simulink model "F90_XMED_03"  (R2025a)
settings: Solver=VariableStepAuto  StartTime=0.0  StopTime=24  RelTol=1e-3
model workspace (MATLAB code in the model file):
  | v_M_exhale = 490; % cmH2O (PEEP)
  | v_M_inhale = 1471; % (PIP)
  | R_M = 0; %
  | 
  | R_V1 = 5670; % cmH2O/L/s
  | R_V2 = 5670;
  | R_I1 = 5670; % tube length = 1.8 ms
  | R_I2 = 5670;
  | R_EV1 = 0;
  | R_EV2 = 0;
  | 
  | R_L1 = 196133;
  | R_L2 = 196133;
  | C_L1 = 5.50647e-7; % L/cmH2O
  | C_L2 = 5.50647e-7;
  | R_ETT1 = 784000;
  | R_ETT2 = 784000;
  | 
  | % === artificial patients (bags)s ====
  | R_aL1 = 196133;
  | R_aL2 = 196133;
  | C_aL1 = 5.50647e-7;
  | C_aL2 = 5.50647e-7;
  | % =======
  | 
  | R_E1 = 5670;
  | R_E2 = 5670;
  | R_O = 0;
  | 
  | RR = 15;
  | I = 1;
  | E = 2;
  | IE_ratio = I/ E;
undefined symbols (not defined in the file): max_inspiratory_pressure_cmH2O, patient1_compliance_L_per_cmH2O, patient1_resistance_cmH2O_per_Lps, patient2_compliance_L_per_cmH2O, patient2_resistance_cmH2O_per_Lps, peep_cmH2O, respiratory_rate_bpm, target_step_time_s, target_tv1_final_mL, target_tv1_initial_mL, target_tv2_final_mL, target_tv2_initial_mL
libraries: fl_lib x39, nesl_utility x16
settings Model: Creator=jsolislemus  LastModifiedBy=SimuVerity Contributors
settings SolverCC: AlgebraicLoopSolver=TrustRegion
settings DataIOCC: SignalLogging=off
settings DebuggingCC: UnconnectedInputMsg=warning  UnconnectedOutputMsg=warning  UnconnectedLineMsg=warning
settings ModelReferenceCC: EnableRefExpFcnMdlSchedulingChecks=on
settings RTWCC: GPUComputeCapability=3.5

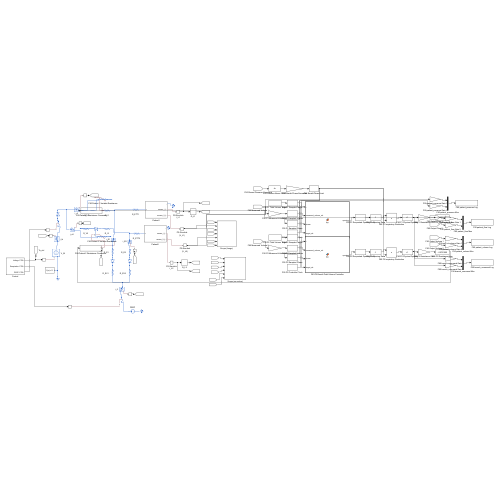
[thumbnail: Simulink's stored preview of the top-level diagram]
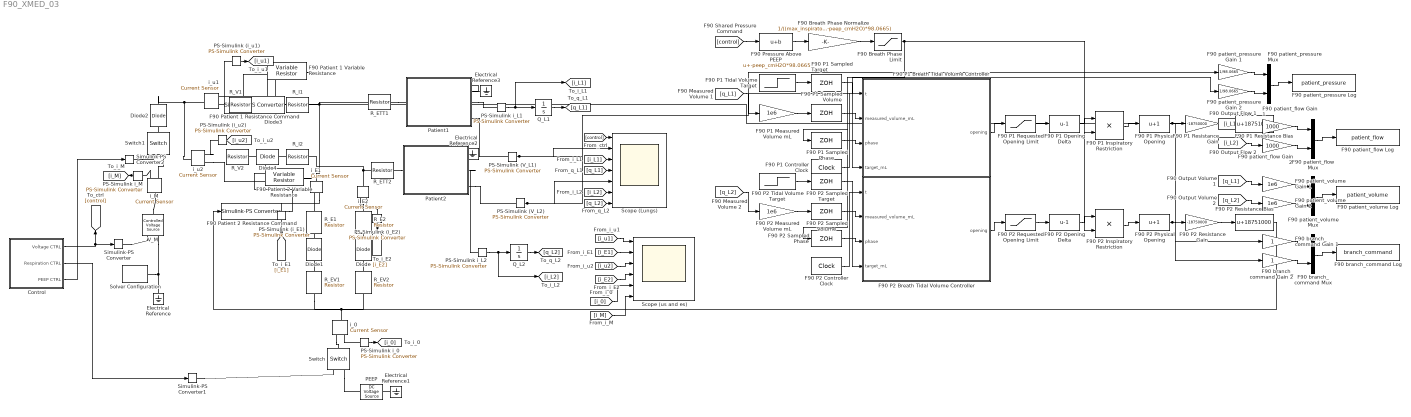
== system F90_XMED_03 ==
  Control : Subsystem
  Diode{,1..4} (5 alike) : fl_lib/Electrical/Electrical Elements/Diode  Vf=0.6 V  Ron=0.3 Ohm  Goff=1e-8 1/Ohm  i_specify=off  i_priority=None  i=0 A  i_nominal_specify=off  i_nominal_value=1  i_nominal_unit=A  v_specify=off  v_priority=None  v=0 V  v_nominal_specify=off  v_nominal_value=1  v_nominal_unit=V
  Electrical Reference{,1..3} (4 alike) : fl_lib/Electrical/Electrical Elements/Electrical Reference
  F90 Breath Phase Limit : Saturate  UpperLimit=1  LowerLimit=0
  F90 Breath Phase Normalize : Gain  Gain=1/((max_inspiratory_pressure_cmH2O-peep_cmH2O)*98.0665)
  F90 P1 Breath Tidal Volume Controller : MATLAB Function  TreatAsAtomicUnit=on
  F90 P1 Controller Clock : DigitalClock  SampleTime=0.005
  F90 P1 Inspiratory Restriction : Product  Inputs=**
  F90 P1 Measured Volume mL : Gain  Gain=1e6
  F90 P1 Opening Delta : Bias  Bias=-1  SaturateOnIntegerOverflow=off
  F90 P1 Physical Opening : Bias  Bias=1  SaturateOnIntegerOverflow=off
  F90 P1 Requested Opening Limit : Saturate  UpperLimit=1  LowerLimit=0.02
  F90 P1 Resistance Bias : Bias  Bias=18751000  SaturateOnIntegerOverflow=off
  F90 P1 Resistance Gain : Gain  Gain=-18750000
  F90 P1 Sampled Phase : ZeroOrderHold  SampleTime=0.005
  F90 P1 Sampled Target : ZeroOrderHold  SampleTime=0.005
  F90 P1 Sampled Volume : ZeroOrderHold  SampleTime=0.005
  F90 P1 Tidal Volume Target : Step  Time=target_step_time_s  Before=target_tv1_initial_mL  After=target_tv1_final_mL  SampleTime=0
  F90 P2 Breath Tidal Volume Controller : MATLAB Function  TreatAsAtomicUnit=on
  F90 P2 Controller Clock : DigitalClock  SampleTime=0.005
  F90 P2 Inspiratory Restriction : Product  Inputs=**
  F90 P2 Measured Volume mL : Gain  Gain=1e6
  F90 P2 Opening Delta : Bias  Bias=-1  SaturateOnIntegerOverflow=off
  F90 P2 Physical Opening : Bias  Bias=1  SaturateOnIntegerOverflow=off
  F90 P2 Requested Opening Limit : Saturate  UpperLimit=1  LowerLimit=0.02
  F90 P2 Resistance Bias : Bias  Bias=18751000  SaturateOnIntegerOverflow=off
  F90 P2 Resistance Gain : Gain  Gain=-18750000
  F90 P2 Sampled Phase : ZeroOrderHold  SampleTime=0.005
  F90 P2 Sampled Target : ZeroOrderHold  SampleTime=0.005
  F90 P2 Sampled Volume : ZeroOrderHold  SampleTime=0.005
  F90 P2 Tidal Volume Target : Step  Time=target_step_time_s  Before=target_tv2_initial_mL  After=target_tv2_final_mL  SampleTime=0
  F90 Patient 1 Resistance Command : nesl_utility/Simulink-PS Converter  PhysicalDomain=network_engine_domain  SubClassName=ps_input  LeftPortType=input  RightPortType=output  PseudoPeriodic=off  Frequencies=[]  NoiseDistribution=none  NoiseParameters=[]  Unit=Ohm  AffineConversion=off  FilteringAndDerivatives=filter  SimscapeFilterOrder=1  InputFilterTimeConstant=0.002  UdotUserProvided=0
  F90 Patient 1 Variable Resistance : fl_lib/Electrical/Electrical Elements/Variable Resistor  Rmin=1 Ohm  thermalEnable=false  thermal_mass=1 J/K  i_specify=off  i_priority=None  i=0 A  i_nominal_specify=off  i_nominal_value=1  i_nominal_unit=A  v_specify=off  v_priority=None  v=0 V  v_nominal_specify=off  v_nominal_value=1  v_nominal_unit=V  T_specify=off  T_priority=None  T=300 K  T_nominal_specify=off  T_nominal_value=1  T_nominal_unit=K
  F90 Patient 2 Resistance Command : nesl_utility/Simulink-PS Converter  PhysicalDomain=network_engine_domain  SubClassName=ps_input  LeftPortType=input  RightPortType=output  PseudoPeriodic=off  Frequencies=[]  NoiseDistribution=none  NoiseParameters=[]  Unit=Ohm  AffineConversion=off  FilteringAndDerivatives=filter  SimscapeFilterOrder=1  InputFilterTimeConstant=0.002  UdotUserProvided=0
  F90 Patient 2 Variable Resistance : fl_lib/Electrical/Electrical Elements/Variable Resistor  Rmin=1 Ohm  thermalEnable=false  thermal_mass=1 J/K  i_specify=off  i_priority=None  i=0 A  i_nominal_specify=off  i_nominal_value=1  i_nominal_unit=A  v_specify=off  v_priority=None  v=0 V  v_nominal_specify=off  v_nominal_value=1  v_nominal_unit=V  T_specify=off  T_priority=None  T=300 K  T_nominal_specify=off  T_nominal_value=1  T_nominal_unit=K
  F90 Pressure Above PEEP : Bias  Bias=-peep_cmH2O*98.0665  SaturateOnIntegerOverflow=off
  F90 branch_command Gain 1 : Gain
  F90 branch_command Gain 2 : Gain
  F90 branch_command Log : ToWorkspace  VariableName=branch_command  SaveFormat=Timeseries  SampleTime=-1
  F90 branch_command Mux : Mux  Inputs=2
  F90 patient_flow Gain 1 : Gain  Gain=1000
  F90 patient_flow Gain 2 : Gain  Gain=1000
  F90 patient_flow Log : ToWorkspace  VariableName=patient_flow  SaveFormat=Timeseries  SampleTime=-1
  F90 patient_flow Mux : Mux  Inputs=2
  F90 patient_pressure Gain 1 : Gain  Gain=1/98.0665
  F90 patient_pressure Gain 2 : Gain  Gain=1/98.0665
  F90 patient_pressure Log : ToWorkspace  VariableName=patient_pressure  SaveFormat=Timeseries  SampleTime=-1
  F90 patient_pressure Mux : Mux  Inputs=2
  F90 patient_volume Gain 1 : Gain  Gain=1e6
  F90 patient_volume Gain 2 : Gain  Gain=1e6
  F90 patient_volume Log : ToWorkspace  VariableName=patient_volume  SaveFormat=Timeseries  SampleTime=-1
  F90 patient_volume Mux : Mux  Inputs=2
  PEEP : fl_lib/Electrical/Electrical Sources/DC Voltage Source  v0=v_M_exhale V
  PS-Simulink (V_L1) : nesl_utility/PS-Simulink Converter  PhysicalDomain=network_engine_domain  SubClassName=ps_output  LeftPortType=input  RightPortType=output  PseudoPeriodic=off  Frequencies=[]  VectorFormat=1-D array  Unit=inherit  AffineConversion=off
  PS-Simulink (V_L2) : nesl_utility/PS-Simulink Converter  PhysicalDomain=network_engine_domain  SubClassName=ps_output  LeftPortType=input  RightPortType=output  PseudoPeriodic=off  Frequencies=[]  VectorFormat=1-D array  Unit=inherit  AffineConversion=off
  PS-Simulink (i_E1) : nesl_utility/PS-Simulink Converter  PhysicalDomain=network_engine_domain  SubClassName=ps_output  LeftPortType=input  RightPortType=output  PseudoPeriodic=off  Frequencies=[]  VectorFormat=1-D array  Unit=inherit  AffineConversion=off
  PS-Simulink (i_E2) : nesl_utility/PS-Simulink Converter  PhysicalDomain=network_engine_domain  SubClassName=ps_output  LeftPortType=input  RightPortType=output  PseudoPeriodic=off  Frequencies=[]  VectorFormat=1-D array  Unit=inherit  AffineConversion=off
  PS-Simulink (i_u1) : nesl_utility/PS-Simulink Converter  PhysicalDomain=network_engine_domain  SubClassName=ps_output  LeftPortType=input  RightPortType=output  PseudoPeriodic=off  Frequencies=[]  VectorFormat=1-D array  Unit=inherit  AffineConversion=off
  PS-Simulink (i_u2) : nesl_utility/PS-Simulink Converter  PhysicalDomain=network_engine_domain  SubClassName=ps_output  LeftPortType=input  RightPortType=output  PseudoPeriodic=off  Frequencies=[]  VectorFormat=1-D array  Unit=inherit  AffineConversion=off
  PS-Simulink i_0 : nesl_utility/PS-Simulink Converter  PhysicalDomain=network_engine_domain  SubClassName=ps_output  LeftPortType=input  RightPortType=output  PseudoPeriodic=off  Frequencies=[]  VectorFormat=1-D array  Unit=inherit  AffineConversion=off
  PS-Simulink i_L1 : nesl_utility/PS-Simulink Converter  PhysicalDomain=network_engine_domain  SubClassName=ps_output  LeftPortType=input  RightPortType=output  PseudoPeriodic=off  Frequencies=[]  VectorFormat=1-D array  Unit=inherit  AffineConversion=off
  PS-Simulink i_L2 : nesl_utility/PS-Simulink Converter  PhysicalDomain=network_engine_domain  SubClassName=ps_output  LeftPortType=input  RightPortType=output  PseudoPeriodic=off  Frequencies=[]  VectorFormat=1-D array  Unit=inherit  AffineConversion=off
  PS-Simulink i_M : nesl_utility/PS-Simulink Converter  PhysicalDomain=network_engine_domain  SubClassName=ps_output  LeftPortType=input  RightPortType=output  PseudoPeriodic=off  Frequencies=[]  VectorFormat=1-D array  Unit=inherit  AffineConversion=off
  Patient1 : Subsystem
  Patient2 : Subsystem
  Q_L1 : Integrator
  Q_L2 : Integrator
  R_E1 : fl_lib/Electrical/Electrical Elements/Resistor  R=R_E1 Ohm  i_specify=off  i_priority=None  i=0 A  i_nominal_specify=off  i_nominal_value=1  i_nominal_unit=A  v_specify=off  v_priority=None  v=0 V  v_nominal_specify=off  v_nominal_value=1  v_nominal_unit=V
  R_E2 : fl_lib/Electrical/Electrical Elements/Resistor  R=R_E2 Ohm  i_specify=off  i_priority=None  i=0 A  i_nominal_specify=off  i_nominal_value=1  i_nominal_unit=A  v_specify=off  v_priority=None  v=0 V  v_nominal_specify=off  v_nominal_value=1  v_nominal_unit=V
  R_ETT1 : fl_lib/Electrical/Electrical Elements/Resistor  R=R_ETT1 Ohm  i_specify=off  i_priority=None  i=0 A  i_nominal_specify=off  i_nominal_value=1  i_nominal_unit=A  v_specify=off  v_priority=None  v=0 V  v_nominal_specify=off  v_nominal_value=1  v_nominal_unit=V
  R_ETT2 : fl_lib/Electrical/Electrical Elements/Resistor  R=R_ETT2 Ohm  i_specify=off  i_priority=None  i=0 A  i_nominal_specify=off  i_nominal_value=1  i_nominal_unit=A  v_specify=off  v_priority=None  v=0 V  v_nominal_specify=off  v_nominal_value=1  v_nominal_unit=V
  R_EV1 : fl_lib/Electrical/Electrical Elements/Resistor  R=R_EV1 Ohm  i_specify=off  i_priority=None  i=0 A  i_nominal_specify=off  i_nominal_value=1  i_nominal_unit=A  v_specify=off  v_priority=None  v=0 V  v_nominal_specify=off  v_nominal_value=1  v_nominal_unit=V
  R_EV2 : fl_lib/Electrical/Electrical Elements/Resistor  R=R_EV2 Ohm  i_specify=off  i_priority=None  i=0 A  i_nominal_specify=off  i_nominal_value=1  i_nominal_unit=A  v_specify=off  v_priority=None  v=0 V  v_nominal_specify=off  v_nominal_value=1  v_nominal_unit=V
  R_I1 : fl_lib/Electrical/Electrical Elements/Resistor  R=R_I1 Ohm  i_specify=off  i_priority=None  i=0 A  i_nominal_specify=off  i_nominal_value=1  i_nominal_unit=A  v_specify=off  v_priority=None  v=0 V  v_nominal_specify=off  v_nominal_value=1  v_nominal_unit=V
  R_I2 : fl_lib/Electrical/Electrical Elements/Resistor  R=R_I2 Ohm  i_specify=off  i_priority=None  i=0 A  i_nominal_specify=off  i_nominal_value=1  i_nominal_unit=A  v_specify=off  v_priority=None  v=0 V  v_nominal_specify=off  v_nominal_value=1  v_nominal_unit=V
  R_V1 : fl_lib/Electrical/Electrical Elements/Resistor  R=R_V1 Ohm  i_specify=off  i_priority=None  i=0 A  i_nominal_specify=off  i_nominal_value=1  i_nominal_unit=A  v_specify=off  v_priority=None  v=0 V  v_nominal_specify=off  v_nominal_value=1  v_nominal_unit=V
  R_V2 : fl_lib/Electrical/Electrical Elements/Resistor  R=R_V2 Ohm  i_specify=off  i_priority=None  i=0 A  i_nominal_specify=off  i_nominal_value=1  i_nominal_unit=A  v_specify=off  v_priority=None  v=0 V  v_nominal_specify=off  v_nominal_value=1  v_nominal_unit=V
  Scope (Lungs) : Scope  NumInputPorts=7
      settings: ActiveDisplayYMinimum=306.25  ActiveDisplayYMaximum=2143.75
  Scope (us and es) : Scope  NumInputPorts=6
      settings: ActiveDisplayYMinimum=-0.00219  ActiveDisplayYMaximum=0.02286  DataLoggingVariableName=ScopeAdvanced
  Simulink-PS Converter : nesl_utility/Simulink-PS Converter  PhysicalDomain=network_engine_domain  SubClassName=ps_input  LeftPortType=input  RightPortType=output  PseudoPeriodic=off  Frequencies=[]  NoiseDistribution=none  NoiseParameters=[]  Unit=1  AffineConversion=off  FilteringAndDerivatives=provide  SimscapeFilterOrder=1  InputFilterTimeConstant=0.001  UdotUserProvided=0
  Simulink-PS Converter1 : nesl_utility/Simulink-PS Converter  PhysicalDomain=network_engine_domain  SubClassName=ps_input  LeftPortType=input  RightPortType=output  PseudoPeriodic=off  Frequencies=[]  NoiseDistribution=none  NoiseParameters=[]  Unit=1  AffineConversion=off  FilteringAndDerivatives=provide  SimscapeFilterOrder=1  InputFilterTimeConstant=0.001  UdotUserProvided=0
  Simulink-PS Converter2 : nesl_utility/Simulink-PS Converter  PhysicalDomain=network_engine_domain  SubClassName=ps_input  LeftPortType=input  RightPortType=output  PseudoPeriodic=off  Frequencies=[]  NoiseDistribution=none  NoiseParameters=[]  Unit=1  AffineConversion=off  FilteringAndDerivatives=provide  SimscapeFilterOrder=1  InputFilterTimeConstant=0.001  UdotUserProvided=0
  Solver Configuration : nesl_utility/Solver Configuration  PhysicalDomain=network_engine_domain  SubClassName=solver  LeftPortType=input  RightPortType=generic  Tones=[]  Harmonics=[]  SimulateNoise=off  Profile=off  UseLocalSampling=off  EnableSwitchedLinearOptims=on  FrequencyDomain=off  UseCCode=off  RelTol=0.001  AbsTol=1e-06  MinStep=1e-09  ToWorkspace=off  RevertToSquareIcSolve=off  NumHomotopyIterations=100  PhasorMode=off  PhasorModeNumHarmonics=1  ConsistencySolver=NEWTON_FTOL  IndexReductionMethod=DerivativeReplacement  DoDC=off  ResidualTolerance=1e-09  ConsistencyTolSource=GLOBAL  ConsistencyAbsTol=0.001  ConsistencyRelTol=0.001  ConsistencyTolFactor=0.001  UseLocalSolver=off  LocalSolverChoice=NE_BACKWARD_EULER_ADVANCER  ResolveIndetEquations=on  FunctionEvalNumThread=1  LocalSolverSampleTime=0.001  DoFixedCost=off  MaxNonlinIter=3  MaxModeIter=2  ComputeImpulses=off  ImpulseIterations=2  LinearAlgebra=auto  LinearAlgebraNumThread=0  EquationFormulation=NE_TIME_EF  DelaysMemoryBudget=1024  AutomaticFiltering=on  FilteringTimeConstant=0.001  PartitionStorageMethod=AS_NEEDED  PartitionMemoryBudget=1024  PartitionMethod=ROBUST  MultibodyUseLocalSolver=off  MultibodyLocalSolverChoice=ODE1  MultibodyLocalSolverSampleTime=0.001
  Switch : fl_lib/Electrical/Electrical Elements/Switch  R_closed=0.01 Ohm  G_open=1e-8 1/Ohm  Threshold=0.5  i_specify=off  i_priority=None  i=0 A  i_nominal_specify=off  i_nominal_value=1  i_nominal_unit=A  v_specify=off  v_priority=None  v=0 V  v_nominal_specify=off  v_nominal_value=1  v_nominal_unit=V
  Switch1 : fl_lib/Electrical/Electrical Elements/Switch  R_closed=0.01 Ohm  G_open=1e-8 1/Ohm  Threshold=0.5  i_specify=off  i_priority=None  i=0 A  i_nominal_specify=off  i_nominal_value=1  i_nominal_unit=A  v_specify=off  v_priority=None  v=0 V  v_nominal_specify=off  v_nominal_value=1  v_nominal_unit=V
  V_M : fl_lib/Electrical/Electrical Sources/Controlled Voltage Source
  i_0 : fl_lib/Electrical/Electrical Sensors/Current Sensor
  i_E1 : fl_lib/Electrical/Electrical Sensors/Current Sensor
  i_E2 : fl_lib/Electrical/Electrical Sensors/Current Sensor
  i_M : fl_lib/Electrical/Electrical Sensors/Current Sensor
  i_u1 : fl_lib/Electrical/Electrical Sensors/Current Sensor
  i_u2 : fl_lib/Electrical/Electrical Sensors/Current Sensor
  wires:
  PS-Simulink i_L1/1 -> [i_L1], Q_L1/1
  PS-Simulink i_L2/1 -> [i_L2], Q_L2/1
  Q_L1/1 -> [q_L1]
  Q_L2/1 -> [q_L2]
  PS-Simulink (i_u1)/1 -> [i_u1]
  [i_u1] -> Scope (us and es)/1
  [i_u2] -> Scope (us and es)/3
  PS-Simulink (i_u2)/1 -> [i_u2]
  [i_E1] -> Scope (us and es)/2
  [i_E2] -> Scope (us and es)/4
  PS-Simulink (i_E2)/1 -> [i_E2]
  [i_0] -> Scope (us and es)/5
  PS-Simulink i_0/1 -> [i_0]
  PS-Simulink i_M/1 -> [i_M]
  [i_M] -> Scope (us and es)/6
  PS-Simulink (i_E1)/1 -> [i_E1]
  [control] -> Scope (Lungs)/1
  [q_L2] -> Scope (Lungs)/7
  [i_L2] -> Scope (Lungs)/6
  [q_L1] -> Scope (Lungs)/4
  PS-Simulink (V_L1)/1 -> Scope (Lungs)/2, F90 patient_pressure Gain 1/1
  PS-Simulink (V_L2)/1 -> Scope (Lungs)/5, F90 patient_pressure Gain 2/1
  [i_L1] -> Scope (Lungs)/3
  Control/1(Voltage CTRL) -> [control], Simulink-PS Converter/1
  Control/2(Respiration CTRL) -> Simulink-PS Converter1/1
  Control/3(PEEP CTRL) -> Simulink-PS Converter2/1
  [control] -> F90 Pressure Above PEEP/1
  F90 Pressure Above PEEP/1 -> F90 Breath Phase Normalize/1
  F90 Breath Phase Normalize/1 -> F90 Breath Phase Limit/1
  [q_L1] -> F90 P1 Measured Volume mL/1
  F90 P1 Measured Volume mL/1 -> F90 P1 Sampled Volume/1
  F90 Breath Phase Limit/1 -> F90 P1 Sampled Phase/1, F90 P1 Inspiratory Restriction/2, F90 P2 Sampled Phase/1, F90 P2 Inspiratory Restriction/2
  F90 P1 Tidal Volume Target/1 -> F90 P1 Sampled Target/1
  F90 P1 Controller Clock/1 -> F90 P1 Breath Tidal Volume Controller/1(t)
  F90 P1 Sampled Volume/1 -> F90 P1 Breath Tidal Volume Controller/2(measured_volume_mL)
  F90 P1 Sampled Phase/1 -> F90 P1 Breath Tidal Volume Controller/3(phase)
  F90 P1 Sampled Target/1 -> F90 P1 Breath Tidal Volume Controller/4(target_mL)
  F90 P1 Breath Tidal Volume Controller/1(opening) -> F90 P1 Requested Opening Limit/1
  F90 P1 Requested Opening Limit/1 -> F90 P1 Opening Delta/1
  F90 P1 Opening Delta/1 -> F90 P1 Inspiratory Restriction/1
  F90 P1 Inspiratory Restriction/1 -> F90 P1 Physical Opening/1
  F90 P1 Physical Opening/1 -> F90 P1 Resistance Gain/1, F90 branch_command Gain 1/1
  F90 P1 Resistance Gain/1 -> F90 P1 Resistance Bias/1
  [q_L2] -> F90 P2 Measured Volume mL/1
  F90 P2 Measured Volume mL/1 -> F90 P2 Sampled Volume/1
  F90 P2 Tidal Volume Target/1 -> F90 P2 Sampled Target/1
  F90 P2 Controller Clock/1 -> F90 P2 Breath Tidal Volume Controller/1(t)
  F90 P2 Sampled Volume/1 -> F90 P2 Breath Tidal Volume Controller/2(measured_volume_mL)
  F90 P2 Sampled Phase/1 -> F90 P2 Breath Tidal Volume Controller/3(phase)
  F90 P2 Sampled Target/1 -> F90 P2 Breath Tidal Volume Controller/4(target_mL)
  F90 P2 Breath Tidal Volume Controller/1(opening) -> F90 P2 Requested Opening Limit/1
  F90 P2 Requested Opening Limit/1 -> F90 P2 Opening Delta/1
  F90 P2 Opening Delta/1 -> F90 P2 Inspiratory Restriction/1
  F90 P2 Inspiratory Restriction/1 -> F90 P2 Physical Opening/1
  F90 P2 Physical Opening/1 -> F90 P2 Resistance Gain/1, F90 branch_command Gain 2/1
  F90 P2 Resistance Gain/1 -> F90 P2 Resistance Bias/1
  F90 P1 Resistance Bias/1 -> F90 Patient 1 Resistance Command/1
  F90 P2 Resistance Bias/1 -> F90 Patient 2 Resistance Command/1
  F90 patient_pressure Gain 1/1 -> F90 patient_pressure Mux/1
  F90 patient_pressure Gain 2/1 -> F90 patient_pressure Mux/2
  F90 patient_pressure Mux/1 -> F90 patient_pressure Log/1
  [i_L1] -> F90 patient_flow Gain 1/1
  [i_L2] -> F90 patient_flow Gain 2/1
  F90 patient_flow Gain 1/1 -> F90 patient_flow Mux/1
  F90 patient_flow Gain 2/1 -> F90 patient_flow Mux/2
  F90 patient_flow Mux/1 -> F90 patient_flow Log/1
  [q_L1] -> F90 patient_volume Gain 1/1
  [q_L2] -> F90 patient_volume Gain 2/1
  F90 patient_volume Gain 1/1 -> F90 patient_volume Mux/1
  F90 patient_volume Gain 2/1 -> F90 patient_volume Mux/2
  F90 patient_volume Mux/1 -> F90 patient_volume Log/1
  F90 branch_command Gain 1/1 -> F90 branch_command Mux/1
  F90 branch_command Gain 2/1 -> F90 branch_command Mux/2
  F90 branch_command Mux/1 -> F90 branch_command Log/1
  connections:
  Simulink-PS Converter/RConn1 -- V_M/RConn1
  V_M/RConn2 -- Solver Configuration/RConn1 -- Electrical Reference/LConn1
  i_u1/LConn1 -- Diode2/RConn1 -- i_u2/LConn1
  R_ETT2/LConn1 -- R_I2/RConn1 -- i_E2/LConn1
  Simulink-PS Converter1/RConn1 -- Switch/RConn1
  i_E2/RConn2 -- R_E2/LConn1
  i_M/LConn1 -- V_M/LConn1
  i_0/RConn2 -- Switch/LConn1
  i_u1/RConn1 -- PS-Simulink (i_u1)/LConn1
  i_u2/RConn1 -- PS-Simulink (i_u2)/LConn1
  i_0/RConn1 -- PS-Simulink i_0/LConn1
  i_E2/RConn1 -- PS-Simulink (i_E2)/LConn1
  i_E1/RConn1 -- PS-Simulink (i_E1)/LConn1
  i_M/RConn1 -- PS-Simulink i_M/LConn1
  Electrical Reference3/LConn1 -- Patient1/RConn1
  Patient1/RConn2 -- PS-Simulink i_L1/LConn1
  Patient1/RConn3 -- PS-Simulink (V_L1)/LConn1
  Electrical Reference2/LConn1 -- Patient2/RConn1
  Patient2/RConn3 -- PS-Simulink (V_L2)/LConn1
  Patient2/RConn2 -- PS-Simulink i_L2/LConn1
  R_E1/LConn1 -- i_E1/RConn2
  R_ETT1/RConn1 -- Patient1/LConn1
  R_ETT1/LConn1 -- i_E1/LConn1 -- R_I1/RConn1
  R_ETT2/RConn1 -- Patient2/LConn1
  Diode/LConn1 -- R_E2/RConn1
  Switch1/LConn1 -- Diode2/LConn1
  Switch1/RConn2 -- i_M/RConn2
  Simulink-PS Converter2/RConn1 -- Switch1/RConn1
  PEEP/RConn1 -- Electrical Reference1/LConn1
  Switch/RConn2 -- PEEP/LConn1
  Diode1/LConn1 -- R_E1/RConn1
  Diode3/LConn1 -- R_V1/RConn1
  Diode3/RConn1 -- R_I1/LConn1
  Diode4/LConn1 -- R_V2/RConn1
  Diode4/RConn1 -- R_I2/LConn1
  R_EV1/LConn1 -- Diode1/RConn1
  R_EV2/LConn1 -- Diode/RConn1
  R_EV1/RConn1 -- R_EV2/RConn1 -- i_0/LConn1
  i_u1/RConn2 -- F90 Patient 1 Variable Resistance/LConn2
  F90 Patient 1 Variable Resistance/RConn1 -- R_V1/LConn1
  F90 Patient 1 Resistance Command/RConn1 -- F90 Patient 1 Variable Resistance/LConn1
  i_u2/RConn2 -- F90 Patient 2 Variable Resistance/LConn2
  F90 Patient 2 Variable Resistance/RConn1 -- R_V2/LConn1
  F90 Patient 2 Resistance Command/RConn1 -- F90 Patient 2 Variable Resistance/LConn1

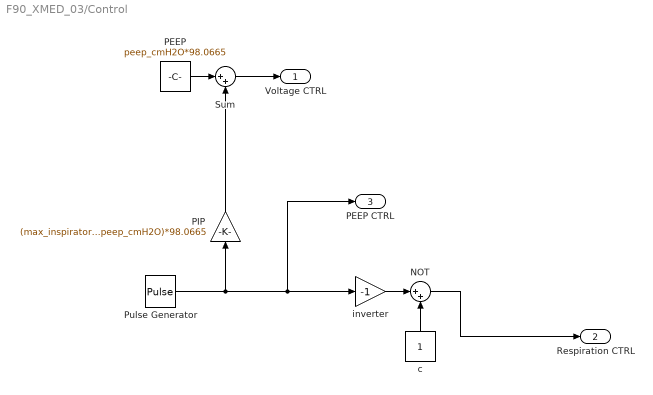
== system F90_XMED_03/Control ==
  NOT : Sum  Inputs=|++
  PEEP : Constant  Value=peep_cmH2O*98.0665
  PIP : Gain  Gain=(max_inspiratory_pressure_cmH2O-peep_cmH2O)*98.0665
  Pulse Generator : DiscretePulseGenerator  PulseType=Time based  Period=60/respiratory_rate_bpm  PulseWidth=IE_ratio/(IE_ratio+1)*100
  Sum : Sum  Inputs=|++
  c : Constant
  inverter : Gain  Gain=-1
  Voltage CTRL : Outport
  Respiration CTRL : Outport  Port=2
  PEEP CTRL : Outport  Port=3
  wires:
  NOT/1 -> Respiration CTRL/1
  Pulse Generator/1 -> PEEP CTRL/1, inverter/1, PIP/1
  inverter/1 -> NOT/1
  Sum/1 -> Voltage CTRL/1
  PEEP/1 -> Sum/1
  PIP/1 -> Sum/2
  c/1 -> NOT/2

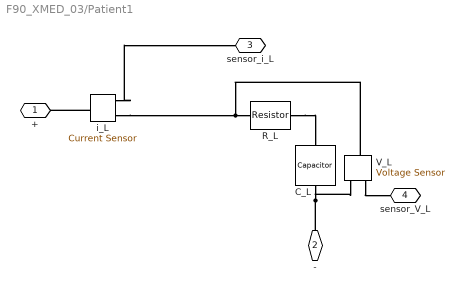
== system F90_XMED_03/Patient1 ==
  C_L : fl_lib/Electrical/Electrical Elements/Capacitor  c=patient1_compliance_L_per_cmH2O*(5.50647e-7/0.054) F  r=1e-6 Ohm  g=0 1/Ohm  i_specify=off  i_priority=None  i=0 A  i_nominal_specify=off  i_nominal_value=1  i_nominal_unit=A  v_specify=off  v_priority=None  v=0 V  v_nominal_specify=off  v_nominal_value=1  v_nominal_unit=V  vc_specify=off  vc_priority=High  vc=0 V  vc_nominal_specify=off  vc_nominal_value=1  vc_nominal_unit=V
  R_L : fl_lib/Electrical/Electrical Elements/Resistor  R=patient1_resistance_cmH2O_per_Lps*98066.5 Ohm  i_specify=off  i_priority=None  i=0 A  i_nominal_specify=off  i_nominal_value=1  i_nominal_unit=A  v_specify=off  v_priority=None  v=0 V  v_nominal_specify=off  v_nominal_value=1  v_nominal_unit=V
  V_L : fl_lib/Electrical/Electrical Sensors/Voltage Sensor
  i_L : fl_lib/Electrical/Electrical Sensors/Current Sensor
  + : PMIOPort  Side=Left
  - : PMIOPort  Port=2  Side=Right
  sensor_i_L : PMIOPort  Port=3  Side=Right
  sensor_V_L : PMIOPort  Port=4  Side=Right
  connections:
  i_L/LConn1 -- +/RConn1
  C_L/RConn1 -- V_L/RConn2 -- -/RConn1
  i_L/RConn1 -- sensor_i_L/RConn1
  V_L/RConn1 -- sensor_V_L/RConn1
  R_L/RConn1 -- C_L/LConn1
  R_L/LConn1 -- i_L/RConn2 -- V_L/LConn1

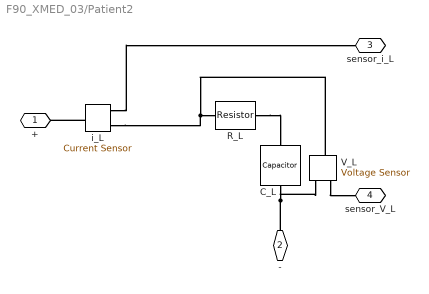
== system F90_XMED_03/Patient2 ==
  C_L : fl_lib/Electrical/Electrical Elements/Capacitor  c=patient2_compliance_L_per_cmH2O*(5.50647e-7/0.054) F  r=1e-6 Ohm  g=0 1/Ohm  i_specify=off  i_priority=None  i=0 A  i_nominal_specify=off  i_nominal_value=1  i_nominal_unit=A  v_specify=off  v_priority=None  v=0 V  v_nominal_specify=off  v_nominal_value=1  v_nominal_unit=V  vc_specify=off  vc_priority=High  vc=0 V  vc_nominal_specify=off  vc_nominal_value=1  vc_nominal_unit=V
  R_L : fl_lib/Electrical/Electrical Elements/Resistor  R=patient2_resistance_cmH2O_per_Lps*98066.5 Ohm  i_specify=off  i_priority=None  i=0 A  i_nominal_specify=off  i_nominal_value=1  i_nominal_unit=A  v_specify=off  v_priority=None  v=0 V  v_nominal_specify=off  v_nominal_value=1  v_nominal_unit=V
  V_L : fl_lib/Electrical/Electrical Sensors/Voltage Sensor
  i_L : fl_lib/Electrical/Electrical Sensors/Current Sensor
  + : PMIOPort  Side=Left
  - : PMIOPort  Port=2  Side=Right
  sensor_i_L : PMIOPort  Port=3  Side=Right
  sensor_V_L : PMIOPort  Port=4  Side=Right
  connections:
  i_L/LConn1 -- +/RConn1
  V_L/RConn2 -- C_L/RConn1 -- -/RConn1
  i_L/RConn1 -- sensor_i_L/RConn1
  V_L/RConn1 -- sensor_V_L/RConn1
  R_L/RConn1 -- C_L/LConn1
  V_L/LConn1 -- i_L/RConn2 -- R_L/LConn1

== matlab function F90_XMED_03/F90 P2 Breath Tidal Volume Controller ==
  data: t input; opening output; measured_volume_mL input; phase input; target_mL input
function opening = fcn(t, measured_volume_mL, phase, target_mL)
%#codegen
persistent previous_phase volume_min
if isempty(previous_phase) || t <= 1e-9
    previous_phase = phase;
    volume_min = measured_volume_mL;
end
if phase <= 0.05
    volume_min = min(volume_min, measured_volume_mL);
    opening = 1;
else
    if previous_phase <= 0.05
    volume_min = measured_volume_mL;
    end
    delivered_mL = max(measured_volume_mL - volume_min, 0);
    remaining_fraction = (target_mL - delivered_mL) / max(target_mL, 1);
    opening = min(max(5*remaining_fraction, 0.02), 1);
end
previous_phase = phase;
end

== matlab function F90_XMED_03/F90 P1 Breath Tidal Volume Controller ==
  data: t input; opening output; measured_volume_mL input; phase input; target_mL input
function opening = fcn(t, measured_volume_mL, phase, target_mL)
%#codegen
persistent previous_phase volume_min
if isempty(previous_phase) || t <= 1e-9
    previous_phase = phase;
    volume_min = measured_volume_mL;
end
if phase <= 0.05
    volume_min = min(volume_min, measured_volume_mL);
    opening = 1;
else
    if previous_phase <= 0.05
    volume_min = measured_volume_mL;
    end
    delivered_mL = max(measured_volume_mL - volume_min, 0);
    remaining_fraction = (target_mL - delivered_mL) / max(target_mL, 1);
    opening = min(max(5*remaining_fraction, 0.02), 1);
end
previous_phase = phase;
end
